simulink model "slide_mode_control"  (R2025b)
settings: Solver=ode23tb  StartTime=0.0  StopTime=t(end)  FixedStep=Ts  RelTol=1e-5
values from neighbouring files (symbols this model uses):
  alpha_0 = 0    [trajectory_smooth.m]
  beta_0 = 0    [trajectory_smooth.m]
  c = 40    [data.m]
  c1_inner = 15.0    (= 15)    [control_params.m]
  c1_outer = 5.0    (= 5)    [control_params.m]
  c1_swing = 8.5    [control_params.m]
  c2_inner = 4.5    [control_params.m]
  c2_outer = 7.5    [control_params.m]
  c2_swing = 5.5    [control_params.m]
  c_plant = c    (= 40)    [data.m]    (also in variation_params.m = scenarios(scen_idx, 2))
  cM = 1.779e-7    (= 1.779e-07)    [data.m]
  cT = 1.105e-5    (= 1.105e-05)    [data.m]
  d = 0.225    [data.m]
  d_alpha_0 = 0    [trajectory_smooth.m]
  d_beta_0 = 0    [trajectory_smooth.m]
  d_l_0 = 0    [trajectory_smooth.m]
  d_phi_0 = 0    [trajectory_smooth.m]
  d_psi_0 = dot_psi_d(1)    [trajectory_smooth.m]
  d_theta_0 = 0    [trajectory_smooth.m]
  d_x_0 = dot_csi_d(1, 1)    [trajectory_smooth.m]
  d_y_0 = dot_csi_d(2, 1)    [trajectory_smooth.m]
  d_z_0 = dot_csi_d(3, 1)    [trajectory_smooth.m]
  delta_val = 0.05    [control_params.m]
  epn_inner = 0.1    [control_params.m]
  epn_outer = 0.1    [control_params.m]
  epn_swing = 0.1    [control_params.m]
  Ixx = 0.0211    [data.m]
  Iyy = Ixx    (= 0.0211)    [data.m]
  Izz = 0.0366    [data.m]
  J_rp = 1.287e-4    (= 0.0001287)    [data.m]
  k = 1e5    (= 100000)    [data.m]
  k_inner = 15.0    (= 15)    [control_params.m]
  k_outer = 2.0    (= 2)    [control_params.m]
  k_plant = k    (= 100000)    [data.m]    (also in variation_params.m = scenarios(scen_idx, 1))
  k_swing = 10.0    (= 10)    [control_params.m]
  l_0 = L_rest + (m_plant*(g+ddot_csi_d(3,1)))/ k_plant    [trajectory_smooth.m]
  L_rest = 1    [data.m]
  M = 2    [data.m]
  m_plant = m    (= 0.5)    [data.m]    (also in variation_params.m = scenarios(scen_idx, 3))
  mu_1_inner = 5/3    (= 1.66666666667)    [control_params.m]
  mu_1_outer = 5/3    (= 1.66666666667)    [control_params.m]
  mu_1_swing = 5/3    (= 1.66666666667)    [control_params.m]
  mu_2_inner = 5/3    (= 1.66666666667)    [control_params.m]
  mu_2_outer = 5/3    (= 1.66666666667)    [control_params.m]
  mu_2_swing = 5/3    (= 1.66666666667)    [control_params.m]
  Omega_0 = w1_0 - w2_0 + w3_0 - w4_0    [trajectory_smooth.m]
  omega_n_1 = 20    [control_params.m]
  omega_n_2 = 20    [control_params.m]
  omega_square_0 = inv(A_alloc) * [u1_hover; u2_hover; u3_hover; u4_hover]    [trajectory_smooth.m]
  phi_0 = 0    [trajectory_smooth.m]
  psi_0 = psi_d(1)    [trajectory_smooth.m]
  theta_0 = 0    [trajectory_smooth.m]
  x_0 = csi_d(1, 1)    [trajectory_smooth.m]
  y_0 = csi_d(2, 1)    [trajectory_smooth.m]
  z_0 = csi_d(3, 1) + l_0    [trajectory_smooth.m]
  zeta_1 = 1    [control_params.m]
  zeta_2 = 1    [control_params.m]
settings Model: Creator=emanu  LastModifiedBy=emanu

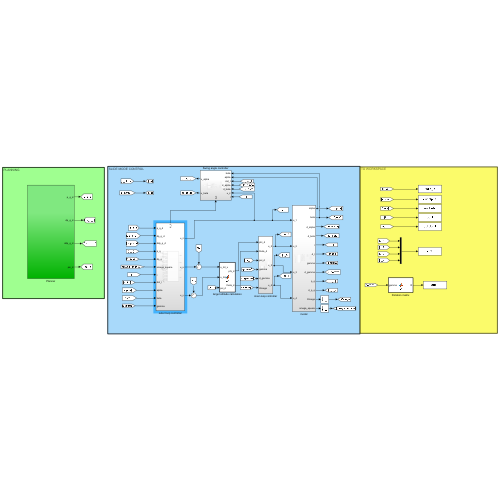
[thumbnail: Simulink's stored preview of the top-level diagram]
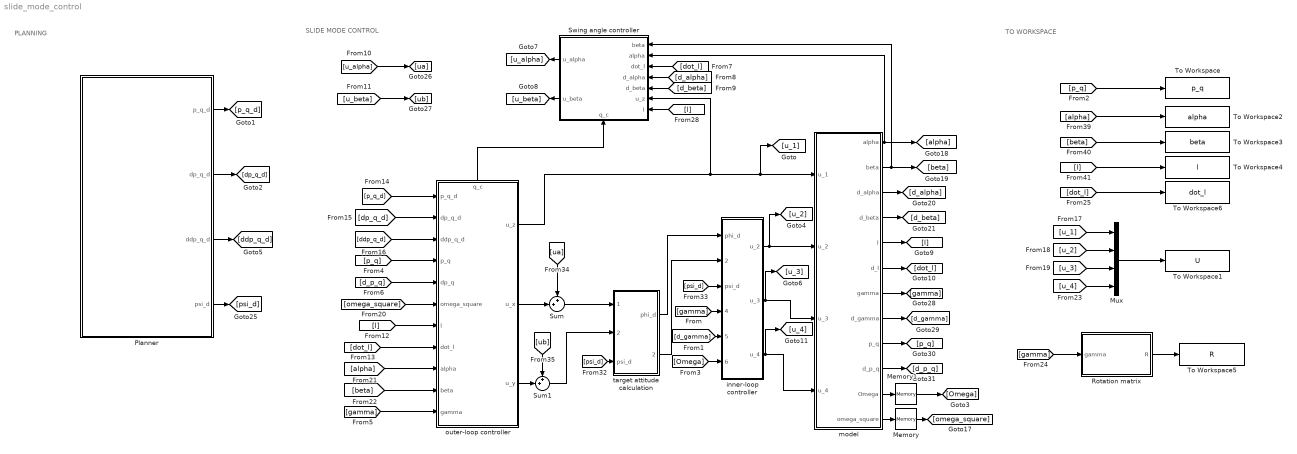
== system slide_mode_control ==
  note: PLANNING
  note: TO WORKSPACE
  note: SLIDE MODE CONTROL
  Memory : Memory  InitialCondition=omega_square_0
  Memory1 : Memory  InitialCondition=Omega_0
  Mux : Mux
  Planner : Subsystem
  Rotation matrix : MATLAB Function  TreatAsAtomicUnit=on
  Sum : Sum  Inputs=++|
  Sum1 : Sum  Inputs=++|
  Swing angle controller : Subsystem
      settings: PortSchema="{\"entries\":[{\"content\":{\"sides\":[{\"content\":{\"connectorIds\":[\"In1\",\"In2\",\"In3\",\"In4\",\"In5\",\"In6\",\"In7\"]},\"type\":\"ConnectorPlacement.EquallySpacedRectSide\",\"uuid\":\"107d9a79-5770-4fe1-afeb-f01ba17b8623\"},{\"content\":{\"connectorIds\":[\"Out1\",\"Out2\"],\"side\":\"RIGHT\"},\"type\":\"ConnectorPlacement.EquallySpacedRectSide\",\"uuid\":\"a16cfd03-53b4-494b-9a38-5d38c3257b94\"},{\"content\":{\"side\":\"TOP\"},\"type\":\"ConnectorPlacement.EquallySpacedRectSide\",\"uuid\":\"c63fb6e7-34b4-45e7-a650-d18239478a3a\"},{\"content\":{\"connectorIds\":[\"In8\"],\"side\":\"BOTTOM\"},\"type\":\"ConnectorPlacement.EquallySpacedRectSide\",\"uuid\":\"a663d818-4b24-4a2f-8491-f9b6658636ee\"}]},\"type\":\"ConnectorPlacement.EquallySpacedConnector\",\"uuid\":\"99174980-2348-474e-adfc-1c682a4a90eb\"}],\"packageUris\":[\"http://schema.mathworks.com/mf0/Connector/R2020b\"],\"version\":\"1.0\"}"
  To Workspace : ToWorkspace  VariableName=p_q  SaveFormat=Timeseries  SampleTime=-1
  To Workspace1 : ToWorkspace  VariableName=U  SaveFormat=Timeseries  SampleTime=-1
  To Workspace2 : ToWorkspace  VariableName=alpha  SaveFormat=Timeseries  SampleTime=-1
  To Workspace3 : ToWorkspace  VariableName=beta  SaveFormat=Timeseries  SampleTime=-1
  To Workspace4 : ToWorkspace  VariableName=l  SaveFormat=Timeseries  SampleTime=-1
  To Workspace5 : ToWorkspace  VariableName=R  SaveFormat=Timeseries  SampleTime=-1
  To Workspace6 : ToWorkspace  VariableName=dot_l  SaveFormat=Timeseries  SampleTime=-1
  inner-loop controller : Subsystem
  model : Subsystem
  outer-loop controller : Subsystem
      settings: PortSchema="{\"entries\":[{\"content\":{\"sides\":[{\"content\":{\"connectorIds\":[\"In1\",\"In2\",\"In3\",\"In4\",\"In5\",\"In6\",\"In7\",\"In8\",\"In9\",\"In10\",\"In11\"]},\"type\":\"ConnectorPlacement.EquallySpacedRectSide\",\"uuid\":\"df6fcbf3-dc8d-434b-9cb1-436330819ec6\"},{\"content\":{\"connectorIds\":[\"Out1\",\"Out2\",\"Out3\"],\"side\":\"RIGHT\"},\"type\":\"ConnectorPlacement.EquallySpacedRectSide\",\"uuid\":\"251502b7-b7f3-4a5f-b6bf-a36f68ad90ea\"},{\"content\":{\"connectorIds\":[\"Out4\"],\"side\":\"TOP\"},\"type\":\"ConnectorPlacement.EquallySpacedRectSide\",\"uuid\":\"43b3d9fa-4196-44c6-9465-37a7290486e2\"}]},\"type\":\"ConnectorPlacement.EquallySpacedConnector\",\"uuid\":\"0c84f21f-ead6-4ba1-8038-c5609232fb5a\"}],\"packageUris\":[\"http://schema.mathworks.com/mf0/Connector/R2020b\"],\"version\":\"1.0\"}"
  target attitude calculation : MATLAB Function  TreatAsAtomicUnit=on
  wires:
  [Omega] -> inner-loop controller/6(Omega)
  outer-loop controller/2(u_x) -> Sum/2
  outer-loop controller/3(u_y) -> Sum1/2
  Swing angle controller/1(u_alpha) -> [u_alpha]
  Swing angle controller/2(u_beta) -> [u_beta]
  Sum1/1 -> target attitude calculation/2(u_tot_y)
  Sum/1 -> target attitude calculation/1(u_tot_x)
  target attitude calculation/2(theta_d) -> inner-loop controller/2(theta_d)
  target attitude calculation/1(phi_d) -> inner-loop controller/1(phi_d)
  inner-loop controller/1(u_2) -> [u_2], model/2(u_2)
  inner-loop controller/2(u_3) -> model/3(u_3), [u_3]
  inner-loop controller/3(u_4) -> model/4(u_4), [u_4]
  outer-loop controller/1(u_z) -> Swing angle controller/6(u_z), [u_1], model/1(u_1)
  Memory/1 -> [omega_square]
  Memory1/1 -> [Omega]
  [dot_l] -> Swing angle controller/3(dot_l)
  [d_alpha] -> Swing angle controller/4(d_alpha)
  [d_beta] -> Swing angle controller/5(d_beta)
  [l] -> Swing angle controller/7(l)
  Planner/4(psi_d) -> [psi_d]
  [psi_d] -> target attitude calculation/3(psi_d)
  [u_beta] -> [ub]
  [u_alpha] -> [ua]
  [ua] -> Sum/1
  [ub] -> Sum1/1
  [beta] -> To Workspace3/1
  [alpha] -> To Workspace2/1
  [l] -> To Workspace4/1
  model/1(alpha) -> Swing angle controller/2(alpha), [alpha]
  model/2(beta) -> Swing angle controller/1(beta), [beta]
  model/3(d_alpha) -> [d_alpha]
  model/4(d_beta) -> [d_beta]
  model/6(d_l) -> [dot_l]
  model/5(l) -> [l]
  model/11(Omega) -> Memory1/1
  model/12(omega_square) -> Memory/1
  model/7(gamma) -> [gamma]
  model/9(p_q) -> [p_q]
  model/10(d_p_q) -> [d_p_q]
  model/8(d_gamma) -> [d_gamma]
  [psi_d] -> inner-loop controller/3(psi_d)
  [gamma] -> inner-loop controller/4(gamma)
  [d_gamma] -> inner-loop controller/5(d_gamma)
  [p_q] -> To Workspace/1
  [omega_square] -> outer-loop controller/6(omega_square)
  [l] -> outer-loop controller/7(l)
  [dot_l] -> outer-loop controller/8(dot_l)
  [alpha] -> outer-loop controller/9(alpha)
  [beta] -> outer-loop controller/10(beta)
  [gamma] -> outer-loop controller/11(gamma)
  [p_q] -> outer-loop controller/4(p_q)
  [d_p_q] -> outer-loop controller/5(dp_q)
  Planner/1(p_q_d) -> [p_q_d]
  [p_q_d] -> outer-loop controller/1(p_q_d)
  Planner/2(dp_q_d) -> [dp_q_d]
  [dp_q_d] -> outer-loop controller/2(dp_q_d)
  Planner/3(ddp_q_d) -> [ddp_q_d]
  [ddp_q_d] -> outer-loop controller/3(ddp_q_d)
  [u_1] -> Mux/1
  [u_2] -> Mux/2
  [u_3] -> Mux/3
  [u_4] -> Mux/4
  Mux/1 -> To Workspace1/1
  [gamma] -> Rotation matrix/1(gamma)
  Rotation matrix/1(R) -> To Workspace5/1
  [dot_l] -> To Workspace6/1
  outer-loop controller/4(q_c) -> Swing angle controller/8(q_c)

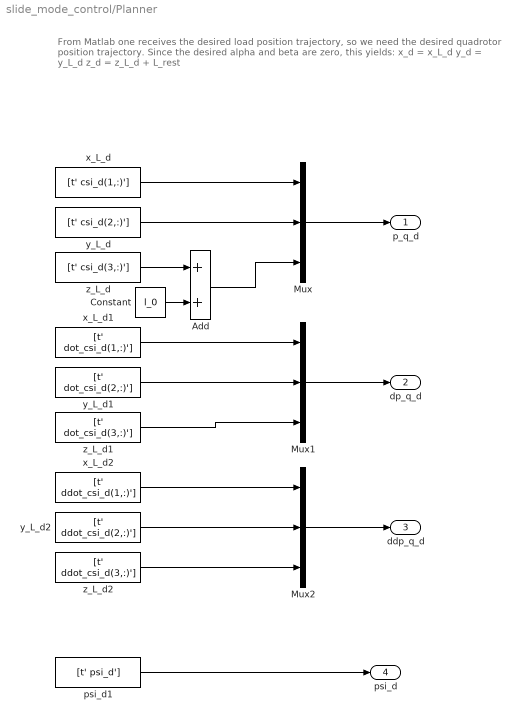
== system slide_mode_control/Planner ==
  note: From Matlab one receives the desired load position trajectory, so we need the desired quadrotor position trajectory. Since the desired alpha and beta are zero, this yields:
      | x_d = x_L_d
      | y_d = y_L_d
      | z_d = z_L_d + L_rest
  Add : Sum
  Constant : Constant  Value=l_0
  Mux : Mux  Inputs=3
  Mux1 : Mux  Inputs=3
  Mux2 : Mux  Inputs=3
  psi_d1 : FromWorkspace  VariableName=[t' psi_d']  OutputAfterFinalValue=Holding final value
  x_L_d : FromWorkspace  VariableName=[t' csi_d(1,:)']  OutputAfterFinalValue=Holding final value
  x_L_d1 : FromWorkspace  VariableName=[t' dot_csi_d(1,:)']  OutputAfterFinalValue=Setting to zero
  x_L_d2 : FromWorkspace  VariableName=[t' ddot_csi_d(1,:)']  OutputAfterFinalValue=Setting to zero
  y_L_d : FromWorkspace  VariableName=[t' csi_d(2,:)']  OutputAfterFinalValue=Holding final value
  y_L_d1 : FromWorkspace  VariableName=[t' dot_csi_d(2,:)']  OutputAfterFinalValue=Setting to zero
  y_L_d2 : FromWorkspace  VariableName=[t' ddot_csi_d(2,:)']  OutputAfterFinalValue=Setting to zero
  z_L_d : FromWorkspace  VariableName=[t' csi_d(3,:)']  OutputAfterFinalValue=Holding final value
  z_L_d1 : FromWorkspace  VariableName=[t' dot_csi_d(3,:)']  OutputAfterFinalValue=Setting to zero
  z_L_d2 : FromWorkspace  VariableName=[t' ddot_csi_d(3,:)']  OutputAfterFinalValue=Holding final value
  p_q_d : Outport
  dp_q_d : Outport  Port=2
  ddp_q_d : Outport  Port=3
  psi_d : Outport  Port=4
  wires:
  z_L_d/1 -> Add/1
  psi_d1/1 -> psi_d/1
  Constant/1 -> Add/2
  Add/1 -> Mux/3
  y_L_d/1 -> Mux/2
  x_L_d/1 -> Mux/1
  Mux/1 -> p_q_d/1
  x_L_d1/1 -> Mux1/1
  y_L_d1/1 -> Mux1/2
  z_L_d2/1 -> Mux2/3
  y_L_d2/1 -> Mux2/2
  x_L_d2/1 -> Mux2/1
  z_L_d1/1 -> Mux1/3
  Mux2/1 -> ddp_q_d/1
  Mux1/1 -> dp_q_d/1

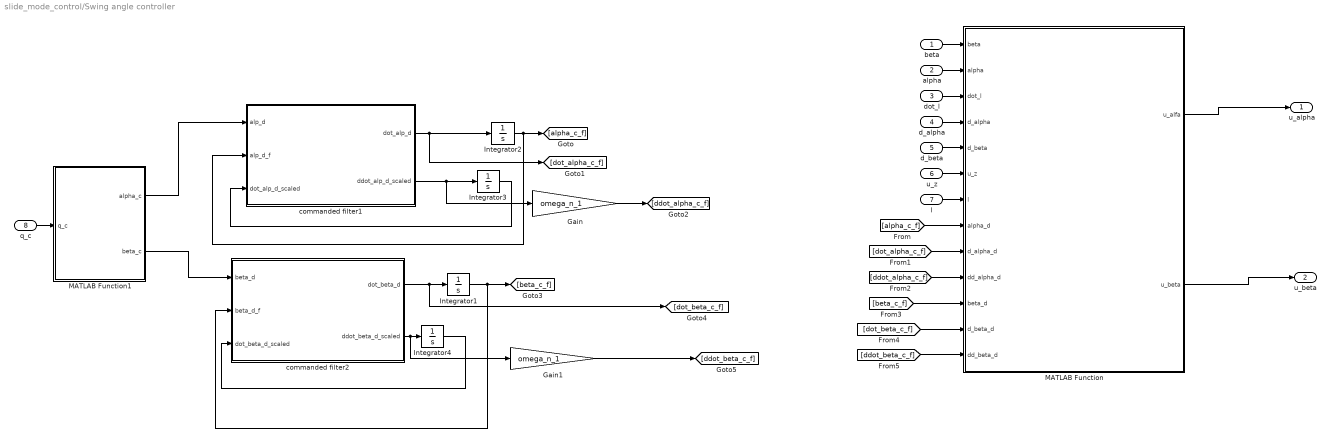
== system slide_mode_control/Swing angle controller ==
  beta : Inport
  alpha : Inport  Port=2
  dot_l : Inport  Port=3
  d_alpha : Inport  Port=4
  d_beta : Inport  Port=5
  u_z : Inport  Port=6
  l : Inport  Port=7
  q_c : Inport  Port=8
  Gain : Gain  Gain=omega_n_1
  Gain1 : Gain  Gain=omega_n_1
  Integrator1 : Integrator  InitialCondition=beta_0
  Integrator2 : Integrator  InitialCondition=alpha_0
  Integrator3 : Integrator  InitialCondition=d_alpha_0
  Integrator4 : Integrator  InitialCondition=d_beta_0
  MATLAB Function : MATLAB Function  TreatAsAtomicUnit=on
  MATLAB Function1 : MATLAB Function  TreatAsAtomicUnit=on
  commanded filter1 : MATLAB Function  TreatAsAtomicUnit=on
  commanded filter2 : MATLAB Function  TreatAsAtomicUnit=on
  u_alpha : Outport
  u_beta : Outport  Port=2
  wires:
  MATLAB Function/1(u_alfa) -> u_alpha/1
  MATLAB Function/2(u_beta) -> u_beta/1
  beta/1 -> MATLAB Function/1(beta)
  alpha/1 -> MATLAB Function/2(alpha)
  dot_l/1 -> MATLAB Function/3(dot_l)
  d_alpha/1 -> MATLAB Function/4(d_alpha)
  d_beta/1 -> MATLAB Function/5(d_beta)
  u_z/1 -> MATLAB Function/6(u_z)
  l/1 -> MATLAB Function/7(l)
  q_c/1 -> MATLAB Function1/1(q_c)
  commanded filter2/1(dot_beta_d) -> [dot_beta_c_f], Integrator1/1
  commanded filter1/1(dot_alp_d) -> [dot_alpha_c_f], Integrator2/1
  commanded filter1/2(ddot_alp_d_scaled) -> Gain/1, Integrator3/1
  Integrator2/1 -> [alpha_c_f], commanded filter1/2(alp_d_f)
  Gain1/1 -> [ddot_beta_c_f]
  Integrator4/1 -> commanded filter2/3(dot_beta_d_scaled)
  commanded filter2/2(ddot_beta_d_scaled) -> Integrator4/1, Gain1/1
  Integrator3/1 -> commanded filter1/3(dot_alp_d_scaled)
  Gain/1 -> [ddot_alpha_c_f]
  MATLAB Function1/1(alpha_c) -> commanded filter1/1(alp_d)
  Integrator1/1 -> [beta_c_f], commanded filter2/2(beta_d_f)
  MATLAB Function1/2(beta_c) -> commanded filter2/1(beta_d)
  [alpha_c_f] -> MATLAB Function/8(alpha_d)
  [dot_alpha_c_f] -> MATLAB Function/9(d_alpha_d)
  [ddot_alpha_c_f] -> MATLAB Function/10(dd_alpha_d)
  [beta_c_f] -> MATLAB Function/11(beta_d)
  [dot_beta_c_f] -> MATLAB Function/12(d_beta_d)
  [ddot_beta_c_f] -> MATLAB Function/13(dd_beta_d)

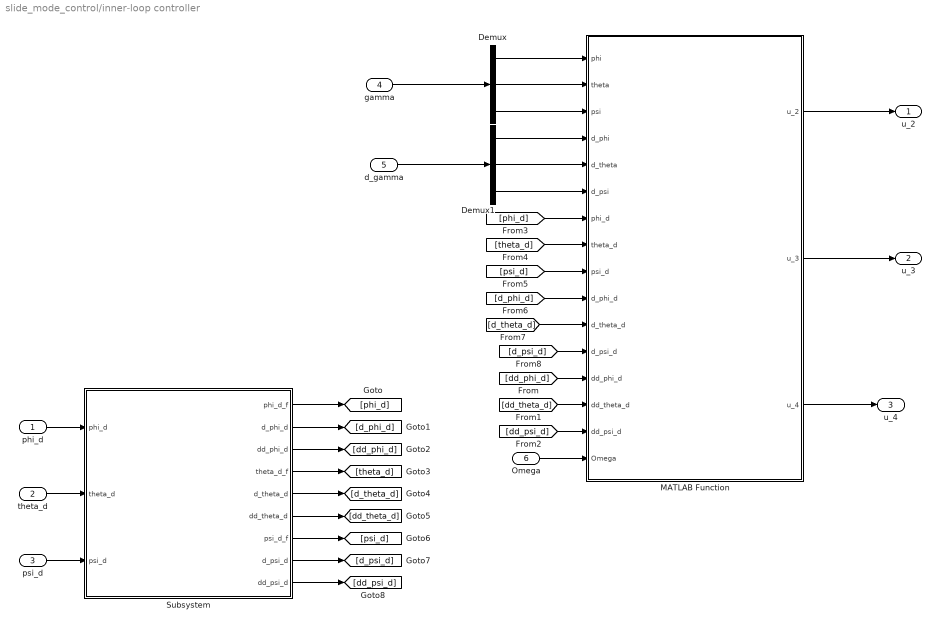
== system slide_mode_control/inner-loop controller ==
  phi_d : Inport
  theta_d : Inport  Port=2
  psi_d : Inport  Port=3
  gamma : Inport  Port=4
  d_gamma : Inport  Port=5
  Omega : Inport  Port=6
  Demux : Demux  Outputs=3
  Demux1 : Demux  Outputs=3
  MATLAB Function : MATLAB Function  TreatAsAtomicUnit=on
  Subsystem : Subsystem
  u_2 : Outport
  u_3 : Outport  Port=2
  u_4 : Outport  Port=3
  wires:
  phi_d/1 -> Subsystem/1(phi_d)
  theta_d/1 -> Subsystem/2(theta_d)
  psi_d/1 -> Subsystem/3(psi_d)
  Subsystem/1(phi_d_f) -> [phi_d]
  Subsystem/2(d_phi_d) -> [d_phi_d]
  Subsystem/3(dd_phi_d) -> [dd_phi_d]
  Subsystem/4(theta_d_f) -> [theta_d]
  Subsystem/5(d_theta_d) -> [d_theta_d]
  Subsystem/6(dd_theta_d) -> [dd_theta_d]
  Subsystem/7(psi_d_f) -> [psi_d]
  Subsystem/8(d_psi_d) -> [d_psi_d]
  Subsystem/9(dd_psi_d) -> [dd_psi_d]
  Omega/1 -> MATLAB Function/16(Omega)
  MATLAB Function/1(u_2) -> u_2/1
  MATLAB Function/2(u_3) -> u_3/1
  MATLAB Function/3(u_4) -> u_4/1
  [dd_phi_d] -> MATLAB Function/13(dd_phi_d)
  [dd_theta_d] -> MATLAB Function/14(dd_theta_d)
  [dd_psi_d] -> MATLAB Function/15(dd_psi_d)
  [d_phi_d] -> MATLAB Function/10(d_phi_d)
  [d_theta_d] -> MATLAB Function/11(d_theta_d)
  [d_psi_d] -> MATLAB Function/12(d_psi_d)
  [phi_d] -> MATLAB Function/7(phi_d)
  [theta_d] -> MATLAB Function/8(theta_d)
  [psi_d] -> MATLAB Function/9(psi_d)
  gamma/1 -> Demux/1
  Demux/1 -> MATLAB Function/1(phi)
  Demux/2 -> MATLAB Function/2(theta)
  Demux/3 -> MATLAB Function/3(psi)
  Demux1/1 -> MATLAB Function/4(d_phi)
  Demux1/2 -> MATLAB Function/5(d_theta)
  Demux1/3 -> MATLAB Function/6(d_psi)
  d_gamma/1 -> Demux1/1

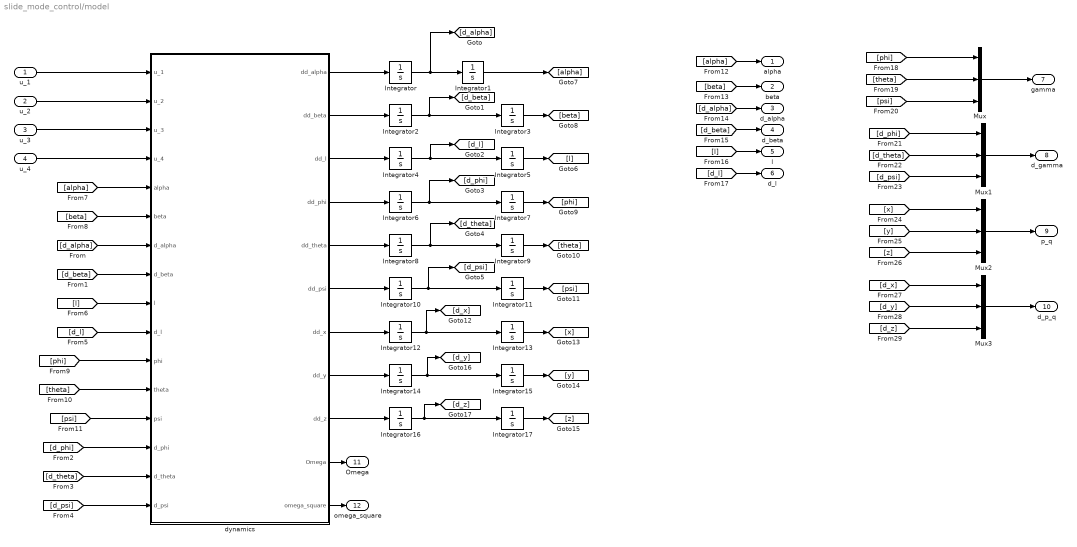
== system slide_mode_control/model ==
  u_1 : Inport
  u_2 : Inport  Port=2
  u_3 : Inport  Port=3
  u_4 : Inport  Port=4
  Integrator : Integrator  InitialCondition=d_alpha_0
  Integrator1 : Integrator  InitialCondition=alpha_0
  Integrator10 : Integrator  InitialCondition=d_psi_0
  Integrator11 : Integrator  InitialCondition=psi_0
  Integrator12 : Integrator  InitialCondition=d_x_0
  Integrator13 : Integrator  InitialCondition=x_0
  Integrator14 : Integrator  InitialCondition=d_y_0
  Integrator15 : Integrator  InitialCondition=y_0
  Integrator16 : Integrator  InitialCondition=d_z_0
  Integrator17 : Integrator  InitialCondition=z_0
  Integrator2 : Integrator  InitialCondition=d_beta_0
  Integrator3 : Integrator  InitialCondition=beta_0
  Integrator4 : Integrator  InitialCondition=d_l_0
  Integrator5 : Integrator  InitialCondition=l_0
  Integrator6 : Integrator  InitialCondition=d_phi_0
  Integrator7 : Integrator  InitialCondition=phi_0
  Integrator8 : Integrator  InitialCondition=d_theta_0
  Integrator9 : Integrator  InitialCondition=theta_0
  Mux{,1..3} (4 alike) : Mux  Inputs=3
  dynamics : MATLAB Function  TreatAsAtomicUnit=on
  alpha : Outport
  beta : Outport  Port=2
  d_alpha : Outport  Port=3
  d_beta : Outport  Port=4
  l : Outport  Port=5
  d_l : Outport  Port=6
  gamma : Outport  Port=7
  d_gamma : Outport  Port=8
  p_q : Outport  Port=9
  d_p_q : Outport  Port=10
  Omega : Outport  Port=11
  omega_square : Outport  Port=12
  wires:
  dynamics/1(dd_alpha) -> Integrator/1
  Integrator/1 -> [d_alpha], Integrator1/1
  dynamics/2(dd_beta) -> Integrator2/1
  Integrator2/1 -> [d_beta], Integrator3/1
  dynamics/3(dd_l) -> Integrator4/1
  dynamics/4(dd_phi) -> Integrator6/1
  dynamics/5(dd_theta) -> Integrator8/1
  Integrator4/1 -> [d_l], Integrator5/1
  Integrator6/1 -> [d_phi], Integrator7/1
  Integrator8/1 -> [d_theta], Integrator9/1
  dynamics/6(dd_psi) -> Integrator10/1
  Integrator10/1 -> [d_psi], Integrator11/1
  dynamics/7(dd_x) -> Integrator12/1
  Integrator12/1 -> [d_x], Integrator13/1
  dynamics/8(dd_y) -> Integrator14/1
  dynamics/9(dd_z) -> Integrator16/1
  Integrator14/1 -> [d_y], Integrator15/1
  Integrator16/1 -> [d_z], Integrator17/1
  [d_alpha] -> dynamics/7(d_alpha)
  [d_beta] -> dynamics/8(d_beta)
  [d_phi] -> dynamics/14(d_phi)
  [d_theta] -> dynamics/15(d_theta)
  [d_psi] -> dynamics/16(d_psi)
  [d_l] -> dynamics/10(d_l)
  Integrator5/1 -> [l]
  [l] -> dynamics/9(l)
  Integrator1/1 -> [alpha]
  Integrator3/1 -> [beta]
  [alpha] -> dynamics/5(alpha)
  [beta] -> dynamics/6(beta)
  u_1/1 -> dynamics/1(u_1)
  u_2/1 -> dynamics/2(u_2)
  u_3/1 -> dynamics/3(u_3)
  u_4/1 -> dynamics/4(u_4)
  Integrator11/1 -> [psi]
  Integrator13/1 -> [x]
  Integrator17/1 -> [z]
  dynamics/10(Omega) -> Omega/1
  dynamics/11(omega_square) -> omega_square/1
  [theta] -> dynamics/12(theta)
  [psi] -> dynamics/13(psi)
  [phi] -> dynamics/11(phi)
  Integrator7/1 -> [phi]
  Integrator9/1 -> [theta]
  Integrator15/1 -> [y]
  [alpha] -> alpha/1
  [beta] -> beta/1
  [d_alpha] -> d_alpha/1
  [d_beta] -> d_beta/1
  [l] -> l/1
  [d_l] -> d_l/1
  [phi] -> Mux/1
  [theta] -> Mux/2
  [psi] -> Mux/3
  Mux/1 -> gamma/1
  Mux1/1 -> d_gamma/1
  [d_psi] -> Mux1/3
  [d_theta] -> Mux1/2
  [d_phi] -> Mux1/1
  [x] -> Mux2/1
  [y] -> Mux2/2
  [z] -> Mux2/3
  Mux2/1 -> p_q/1
  Mux3/1 -> d_p_q/1
  [d_z] -> Mux3/3
  [d_y] -> Mux3/2
  [d_x] -> Mux3/1

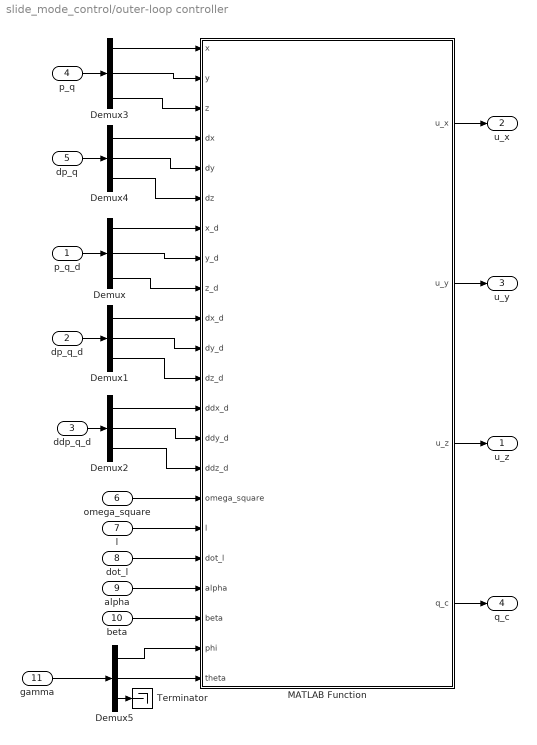
== system slide_mode_control/outer-loop controller ==
  p_q_d : Inport
  dp_q_d : Inport  Port=2
  ddp_q_d : Inport  Port=3
  p_q : Inport  Port=4
  dp_q : Inport  Port=5
  omega_square : Inport  Port=6
  l : Inport  Port=7
  dot_l : Inport  Port=8
  alpha : Inport  Port=9
  beta : Inport  Port=10
  gamma : Inport  Port=11
  Demux{,1..5} (6 alike) : Demux  Outputs=3
  MATLAB Function : MATLAB Function  TreatAsAtomicUnit=on
  Terminator : Terminator
  u_z : Outport
  u_x : Outport  Port=2
  u_y : Outport  Port=3
  q_c : Outport  Port=4
  wires:
  MATLAB Function/1(u_x) -> u_x/1
  MATLAB Function/2(u_y) -> u_y/1
  MATLAB Function/3(u_z) -> u_z/1
  omega_square/1 -> MATLAB Function/16(omega_square)
  l/1 -> MATLAB Function/17(l)
  dot_l/1 -> MATLAB Function/18(dot_l)
  alpha/1 -> MATLAB Function/19(alpha)
  beta/1 -> MATLAB Function/20(beta)
  p_q_d/1 -> Demux/1
  Demux/1 -> MATLAB Function/7(x_d)
  Demux/2 -> MATLAB Function/8(y_d)
  Demux/3 -> MATLAB Function/9(z_d)
  dp_q_d/1 -> Demux1/1
  Demux1/1 -> MATLAB Function/10(dx_d)
  Demux1/2 -> MATLAB Function/11(dy_d)
  Demux1/3 -> MATLAB Function/12(dz_d)
  ddp_q_d/1 -> Demux2/1
  Demux2/1 -> MATLAB Function/13(ddx_d)
  Demux2/2 -> MATLAB Function/14(ddy_d)
  Demux2/3 -> MATLAB Function/15(ddz_d)
  p_q/1 -> Demux3/1
  Demux3/1 -> MATLAB Function/1(x)
  Demux3/2 -> MATLAB Function/2(y)
  Demux3/3 -> MATLAB Function/3(z)
  dp_q/1 -> Demux4/1
  Demux4/1 -> MATLAB Function/4(dx)
  Demux4/2 -> MATLAB Function/5(dy)
  Demux4/3 -> MATLAB Function/6(dz)
  Demux5/3 -> Terminator/1
  gamma/1 -> Demux5/1
  Demux5/1 -> MATLAB Function/21(phi)
  Demux5/2 -> MATLAB Function/22(theta)
  MATLAB Function/4(q_c) -> q_c/1

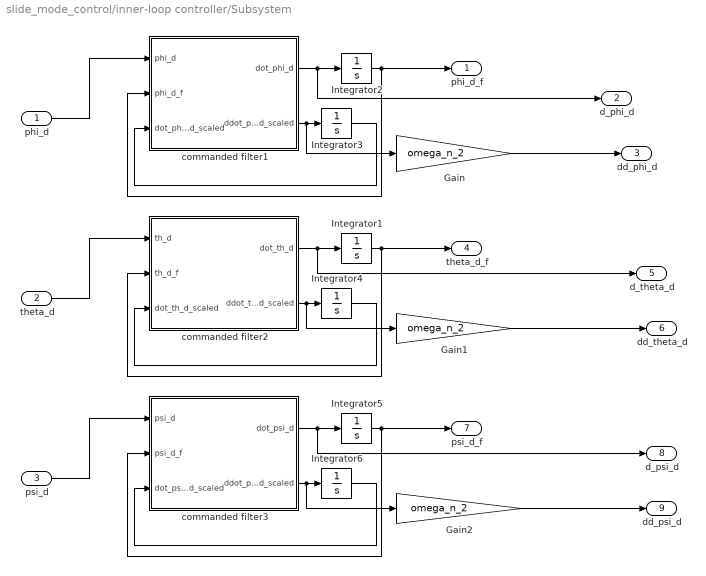
== system slide_mode_control/inner-loop controller/Subsystem ==
  phi_d : Inport
  theta_d : Inport  Port=2
  psi_d : Inport  Port=3
  Gain : Gain  Gain=omega_n_2
  Gain1 : Gain  Gain=omega_n_2
  Gain2 : Gain  Gain=omega_n_2
  Integrator1 : Integrator  InitialCondition=theta_0
  Integrator2 : Integrator  InitialCondition=phi_0
  Integrator3 : Integrator  InitialCondition=d_phi_0
  Integrator4 : Integrator  InitialCondition=d_theta_0
  Integrator5 : Integrator  InitialCondition=psi_0
  Integrator6 : Integrator  InitialCondition=d_psi_0
  commanded filter1 : MATLAB Function  TreatAsAtomicUnit=on
  commanded filter2 : MATLAB Function  TreatAsAtomicUnit=on
  commanded filter3 : MATLAB Function  TreatAsAtomicUnit=on
  phi_d_f : Outport
  d_phi_d : Outport  Port=2
  dd_phi_d : Outport  Port=3
  theta_d_f : Outport  Port=4
  d_theta_d : Outport  Port=5
  dd_theta_d : Outport  Port=6
  psi_d_f : Outport  Port=7
  d_psi_d : Outport  Port=8
  dd_psi_d : Outport  Port=9
  wires:
  phi_d/1 -> commanded filter1/1(phi_d)
  commanded filter1/1(dot_phi_d) -> d_phi_d/1, Integrator2/1
  Integrator2/1 -> phi_d_f/1, commanded filter1/2(phi_d_f)
  Integrator3/1 -> commanded filter1/3(dot_phi_d_scaled)
  commanded filter1/2(ddot_phi_d_scaled) -> Gain/1, Integrator3/1
  Gain/1 -> dd_phi_d/1
  Gain1/1 -> dd_theta_d/1
  commanded filter2/2(ddot_th_d_scaled) -> Gain1/1, Integrator4/1
  Integrator1/1 -> theta_d_f/1, commanded filter2/2(th_d_f)
  Integrator4/1 -> commanded filter2/3(dot_th_d_scaled)
  theta_d/1 -> commanded filter2/1(th_d)
  commanded filter2/1(dot_th_d) -> d_theta_d/1, Integrator1/1
  Gain2/1 -> dd_psi_d/1
  commanded filter3/2(ddot_psi_d_scaled) -> Gain2/1, Integrator6/1
  Integrator5/1 -> psi_d_f/1, commanded filter3/2(psi_d_f)
  Integrator6/1 -> commanded filter3/3(dot_psi_d_scaled)
  psi_d/1 -> commanded filter3/1(psi_d)
  commanded filter3/1(dot_psi_d) -> d_psi_d/1, Integrator5/1

== matlab function slide_mode_control/inner-loop controller/Subsystem/commanded filter2 ==
  data: th_d input; dot_th_d output; th_d_f input; dot_th_d_scaled input; zeta_2 parameter; ddot_th_d_scaled output; omega_n_2 parameter
function [dot_th_d, ddot_th_d_scaled] = fcn(th_d, th_d_f, dot_th_d_scaled, zeta_2, omega_n_2)
    dot_th_d = omega_n_2 * dot_th_d_scaled;
    ddot_th_d_scaled = -2 * zeta_2 * omega_n_2 * dot_th_d_scaled - omega_n_2 * (th_d_f - th_d);
end

== matlab function slide_mode_control/inner-loop controller/Subsystem/commanded filter3 ==
  data: psi_d input; dot_psi_d output; psi_d_f input; dot_psi_d_scaled input; zeta_2 parameter; ddot_psi_d_scaled output; omega_n_2 parameter
function [dot_psi_d, ddot_psi_d_scaled] = fcn(psi_d, psi_d_f, dot_psi_d_scaled, zeta_2, omega_n_2)
    dot_psi_d = omega_n_2 * dot_psi_d_scaled;
    ddot_psi_d_scaled = -2 * zeta_2 * omega_n_2 * dot_psi_d_scaled - omega_n_2 * (psi_d_f - psi_d);
end

== matlab function slide_mode_control/Swing angle controller/MATLAB Function ==
  data: beta input; u_alfa output; u_beta output; alpha input; dot_l input; d_alpha input; d_beta input; u_z input; l input; alpha_d input; d_alpha_d input; dd_alpha_d input; beta_d input; d_beta_d input; dd_beta_d input; M parameter; c1_swing parameter; c2_swing parameter; k_swing parameter; mu_1_swing parameter; mu_2_swing parameter; epn_swing parameter; delta_val parameter
function [u_alfa, u_beta] = fcn(beta, alpha, dot_l, d_alpha, d_beta, u_z, l,alpha_d,d_alpha_d,dd_alpha_d, ...
    beta_d,d_beta_d,dd_beta_d, M,c1_swing, c2_swing,k_swing,mu_1_swing, mu_2_swing, epn_swing, delta_val)
    L = max(l, 1e-3);
    cos_beta = max(cos(beta), 1e-3);
    eps_g = 1e-4;

    g_alfa = -u_z / (M * L * cos_beta);
    g_beta =  -u_z / (M * L);

    f_alfa = -2 * (dot_l * d_alpha / L) + 2 * d_alpha * d_beta * (sin(beta) / cos_beta);
    f_beta = -2 * (dot_l * d_beta / L) - d_alpha^2 * sin(beta) * cos_beta;

    % surface parameters
    c1 = c1_swing; 
    c2 =c2_swing; 
    mu_1 = mu_1_swing; 
    mu_2 = mu_2_swing; 
    epn = epn_swing;

    % Errors
    e_alfa = alpha_d-alpha;
    dot_e_alfa = d_alpha_d-d_alpha;
    e_beta = beta_d-beta;
    dot_e_beta = d_beta_d-d_beta;

  
    s_alfa = e_alfa + c1 * sign(e_alfa) * abs(e_alfa)^mu_1 + c2 * sign(dot_e_alfa) * abs(dot_e_alfa)^mu_2;
    s_beta = e_beta + c1 * sign(e_beta) * abs(e_beta)^mu_1 + c2 * sign(dot_e_beta) * abs(dot_e_beta)^mu_2;

    delta=delta_val;

    num_a = (sign(dot_e_alfa) * abs(dot_e_alfa)^(2-mu_2) / (c2 * mu_2)) * (1 + c1 * mu_1 * abs(e_alfa)^(mu_1-1))+dd_alpha_d- f_alfa + k_swing * s_alfa + epn * sat(s_alfa, delta);
    num_b = (sign(dot_e_beta) * abs(dot_e_beta)^(2-mu_2) / (c2 * mu_2)) * (1 + c1 * mu_1 * abs(e_beta)^(mu_1-1))+dd_beta_d- f_beta + k_swing * s_beta + epn * sat(s_beta, delta);


    if abs(g_alfa) < eps_g
        u_alfa = num_a / (sign(g_alfa + eps) * eps_g);
    else
        u_alfa = num_a / g_alfa;
    end

    if abs(g_beta) < eps_g
        u_beta = num_b / (sign(g_beta + eps) * eps_g);
    else
        u_beta = num_b / g_beta;
    end
end

== matlab function slide_mode_control/outer-loop controller/MATLAB Function ==
  data: u_x output; u_y output; u_z output; x input; y input; z input; dx input; dy input; dz input; x_d input; y_d input; z_d input; dx_d input; dy_d input; dz_d input; ddx_d input; ddy_d input; ddz_d input; omega_square input; k parameter; L_rest parameter; c parameter; l input; dot_l input; alpha input; beta input; M parameter; phi input; theta input; cT parameter; c1_outer parameter; c2_outer parameter; k_outer parameter; mu_1_outer parameter; mu_2_outer parameter; epn_outer parameter; delta_val parameter; q_c output size=3
function [u_x, u_y, u_z,q_c] = fcn(x, y, z, dx, dy, dz,x_d,y_d,z_d,dx_d,dy_d,dz_d, ddx_d, ddy_d, ddz_d, ...
    omega_square, k, L_rest, c, l, dot_l, alpha, beta, M, phi, theta, cT,c1_outer, c2_outer,k_outer, ...
    mu_1_outer, mu_2_outer, epn_outer, delta_val)

T=k*(l-L_rest)+c*dot_l;
Tx=T*sin(alpha)*cos(beta);
Ty=T*sin(beta);
Tz=T*cos(alpha)*cos(beta);
g=9.81;

F=max((cT*sum(omega_square)),1e-3);
cos_phi_theta=max((cos(phi)*cos(theta)), 1e-3);


g_x=F/M;
g_y=g_x;
g_z=cos_phi_theta/M;

f_x=-Tx/M;
f_y=-Ty/M;
f_z=-(Tz/M)-g;

%parameter surface
c1 = c1_outer;
c2 = c2_outer;
mu_1 = mu_1_outer;
mu_2 = mu_2_outer;
epn=epn_outer;

%error
ex=x_d-x;
ey=y_d-y;
ez=z_d-z;
dex=dx_d-dx;
dey=dy_d-dy;
dez=dz_d-dz;

%surface
s_x = ex + c1 * sign(ex) * abs(ex)^mu_1 + c2 * sign(dex) * abs(dex)^mu_2;
s_y = ey + c1 * sign(ey) * abs(ey)^mu_1 + c2 * sign(dey) * abs(dey)^mu_2;
s_z = ez + c1 * sign(ez) * abs(ez)^mu_1 + c2 * sign(dez) * abs(dez)^mu_2;

delta=delta_val;

num_x = (sign(dex) * abs(dex)^(2 - mu_2) / (c2 * mu_2)) * (1 + c1 * mu_1 * abs(ex)^(mu_1 - 1)) + ddx_d - f_x + k_outer * s_x + epn * sat(s_x, delta); 
num_y = (sign(dey) * abs(dey)^(2 - mu_2) / (c2 * mu_2)) * (1 + c1 * mu_1 * abs(ey)^(mu_1 - 1)) + ddy_d - f_y + k_outer * s_y + epn * sat(s_y, delta); 
num_z = (sign(dez) * abs(dez)^(2 - mu_2) / (c2 * mu_2)) * (1 + c1 * mu_1 * abs(ez)^(mu_1 - 1)) + ddz_d - f_z + k_outer * s_z + epn * sat(s_z, delta); 

u_x=num_x/g_x;
u_y=num_y/g_y;
u_z=num_z/g_z;

u_des=[num_x;num_y;num_z];

if norm(u_des)<1e-5
    q_c=[0;0;-1];
else
    q_c=-u_des/norm(u_des);
end

end

== matlab function slide_mode_control/Rotation matrix ==
  data: gamma input; R output
function R = fcn(gamma)

phi=gamma(1);
theta=gamma(2);
psi=gamma(3);

c_phi = cos(phi);   s_phi = sin(phi);
c_the = cos(theta); s_the = sin(theta);
c_psi = cos(psi);   s_psi = sin(psi);

% R_B^E (Z-Y-X Euler angles)
R = [ c_the*c_psi,  s_phi*s_the*c_psi - c_phi*s_psi,  c_phi*s_the*c_psi + s_phi*s_psi;
      c_the*s_psi,  s_phi*s_the*s_psi + c_phi*c_psi,  c_phi*s_the*s_psi - s_phi*c_psi;
     -s_the,        s_phi*c_the,                      c_phi*c_the ];
end

== matlab function slide_mode_control/Swing angle controller/MATLAB Function1 ==
  data: q_c input size=3; alpha_c output; beta_c output
function [alpha_c, beta_c] = fcn(q_c)
    qy = max(min(q_c(2), 1), -1);
    beta_c = asin(qy);
    alpha_c = atan2(q_c(1), -q_c(3));
end

== matlab function slide_mode_control/inner-loop controller/Subsystem/commanded filter1 ==
  data: phi_d input; dot_phi_d output; phi_d_f input; dot_phi_d_scaled input; zeta_2 parameter; ddot_phi_d_scaled output; omega_n_2 parameter
function [dot_phi_d, ddot_phi_d_scaled] = fcn(phi_d, phi_d_f, dot_phi_d_scaled, zeta_2, omega_n_2)
    dot_phi_d = omega_n_2 * dot_phi_d_scaled;
    ddot_phi_d_scaled = -2 * zeta_2 * omega_n_2 * dot_phi_d_scaled - omega_n_2 * (phi_d_f - phi_d);
end

== matlab function slide_mode_control/Swing angle controller/commanded filter1 ==
  data: alp_d input; dot_alp_d output; alp_d_f input; dot_alp_d_scaled input; zeta_1 parameter; ddot_alp_d_scaled output; omega_n_1 parameter
function [dot_alp_d, ddot_alp_d_scaled] = fcn(alp_d, alp_d_f, dot_alp_d_scaled, zeta_1, omega_n_1)
    dot_alp_d = omega_n_1 * dot_alp_d_scaled;
    ddot_alp_d_scaled = -2 * zeta_1 * omega_n_1 * dot_alp_d_scaled - omega_n_1 * (alp_d_f - alp_d);
end

== matlab function slide_mode_control/target attitude calculation ==
  data: u_tot_x input; phi_d output; u_tot_y input; psi_d input; theta_d output
function [phi_d, theta_d] = fcn(u_tot_x, u_tot_y, psi_d)

term_1=sin(psi_d)*u_tot_x-cos(psi_d)*u_tot_y;
term_2=min(max(term_1,-1),1);
phi_d=asin(term_2);

cos_phi=max(cos(phi_d), 1e-3);

term_3=(cos(psi_d) * u_tot_x + sin(psi_d) * u_tot_y) / cos_phi;
term_4=min(max(term_3,-1),1);
theta_d=asin(term_4);
    
   
end

== matlab function slide_mode_control/Swing angle controller/commanded filter2 ==
  data: beta_d input; dot_beta_d output; beta_d_f input; dot_beta_d_scaled input; zeta_2 parameter; ddot_beta_d_scaled output; omega_n_2 parameter
function [dot_beta_d, ddot_beta_d_scaled] = fcn(beta_d, beta_d_f, dot_beta_d_scaled, zeta_2, omega_n_2)
    dot_beta_d = omega_n_2 * dot_beta_d_scaled;
    ddot_beta_d_scaled = -2 * zeta_2 * omega_n_2 * dot_beta_d_scaled - omega_n_2 * (beta_d_f - beta_d);
end

== matlab function slide_mode_control/inner-loop controller/MATLAB Function ==
  data: u_2 output; u_3 output; u_4 output; phi input; theta input; psi input; d_phi input; d_theta input; d_psi input; phi_d input; theta_d input; psi_d input; d_phi_d input; d_theta_d input; d_psi_d input; dd_phi_d input; dd_theta_d input; dd_psi_d input; Omega input; Ixx parameter; J_rp parameter; Iyy parameter; Izz parameter; c1_inner parameter; c2_inner parameter; k_inner parameter; mu_1_inner parameter; mu_2_inner parameter; epn_inner parameter; delta_val parameter
function [u_2, u_3, u_4] = fcn(phi, theta, psi, d_phi, d_theta, d_psi, phi_d, theta_d, psi_d, ...
    d_phi_d, d_theta_d, d_psi_d, dd_phi_d, ...
    dd_theta_d, dd_psi_d, Omega, Ixx, J_rp, Iyy, Izz, c1_inner, c2_inner,k_inner,mu_1_inner,mu_2_inner,epn_inner,delta_val)

    e_phi   = phi_d - phi;
    e_theta = theta_d - theta;
    e_psi   = psi_d - psi;

    dot_e_phi   = d_phi_d - d_phi;
    dot_e_theta = d_theta_d - d_theta;
    dot_e_psi   = d_psi_d - d_psi;

    g_phi   = 1 / Ixx;
    g_theta = 1 / Iyy;
    g_psi   = 1 / Izz;

    f_phi   = d_theta * d_psi * (Iyy - Izz) + J_rp * d_theta * Omega;
    f_theta = d_phi * d_psi * (Izz - Ixx) + J_rp * d_phi * Omega;
    f_psi   = d_phi * d_theta * (Ixx - Iyy);

    % Surface parameters
    c1 = c1_inner; 
    c2 = c2_inner; 
    mu_1 = mu_1_inner; 
    mu_2 = mu_2_inner; 
    epn = epn_inner;


    s_phi   = e_phi   + c1 * sign(e_phi)   * abs(e_phi)^mu_1   + c2 * sign(dot_e_phi)   * abs(dot_e_phi)^mu_2;
    s_theta = e_theta + c1 * sign(e_theta) * abs(e_theta)^mu_1 + c2 * sign(dot_e_theta) * abs(dot_e_theta)^mu_2;
    s_psi   = e_psi   + c1 * sign(e_psi)   * abs(e_psi)^mu_1   + c2 * sign(dot_e_psi)   * abs(dot_e_psi)^mu_2;

    delta=delta_val;

    num2 = (sign(dot_e_phi) * abs(dot_e_phi)^(2-mu_2) / (c2 * mu_2)) * (1 + c1 * mu_1 * abs(e_phi)^(mu_1-1)) + dd_phi_d - f_phi + k_inner * s_phi + epn * sat(s_phi, delta);
    num3 = (sign(dot_e_theta) * abs(dot_e_theta)^(2-mu_2) / (c2 * mu_2)) * (1 + c1 * mu_1 * abs(e_theta)^(mu_1-1)) + dd_theta_d - f_theta + k_inner * s_theta + epn * sat(s_theta, delta);
    num4 = (sign(dot_e_psi) * abs(dot_e_psi)^(2-mu_2) / (c2 * mu_2)) * (1 + c1 * mu_1 * abs(e_psi)^(mu_1-1)) + dd_psi_d - f_psi + k_inner * s_psi + epn * sat(s_psi, delta);

    u_2 = num2 / g_phi;
    u_3 = num3 / g_theta;
    u_4 = num4 / g_psi;
end

== matlab function slide_mode_control/model/dynamics ==
  data: u_1 input; u_2 input; u_3 input; u_4 input; alpha input; beta input; d_alpha input; d_beta input; l input; d_l input; phi input; theta input; psi input; d_phi input; d_theta input; d_psi input; dd_alpha output; dd_beta output; dd_l output; dd_phi output; dd_theta output; dd_psi output; dd_x output; dd_y output; dd_z output; M parameter; k_plant parameter; c_plant parameter; L_rest parameter; m_plant parameter; Ixx parameter; Iyy parameter; Izz parameter; cT parameter; cM parameter; d parameter; J_rp parameter; Omega output; omega_square output
function [dd_alpha,dd_beta,dd_l,dd_phi,dd_theta,dd_psi,dd_x,dd_y,dd_z,Omega, omega_square]=dynamics(u_1,u_2,u_3,u_4,alpha, ...
    beta,d_alpha,d_beta,l,d_l,phi,theta,psi,d_phi,d_theta,d_psi,M, k_plant, c_plant, L_rest, ...
    m_plant, Ixx, Iyy, Izz, cT, cM, d, J_rp)

l_safe = max(l, 0.05);
cos_beta_safe = max(cos(beta), 0.05);
g=9.81;
T=k_plant*(l-L_rest)+c_plant*d_l;
a=sqrt(2)/2;
A=[cT cT cT cT;-a*d*cT a*d*cT a*d*cT -a*d*cT;-a*d*cT -a*d*cT a*d*cT a*d*cT;-cM cM -cM cM];
omega_square= inv(A)*[u_1;u_2;u_3;u_4];
w1 = sqrt(max(0, omega_square(1)));
w2 = sqrt(max(0, omega_square(2)));
w3 = sqrt(max(0, omega_square(3)));
w4 = sqrt(max(0, omega_square(4)));

Omega = w1 - w2 + w3 - w4;

Fx = u_1 * (cos(psi)*sin(theta)*cos(phi) + sin(psi)*sin(phi));
Fy = u_1 * (sin(psi)*sin(theta)*cos(phi) - cos(psi)*sin(phi));
Fz = u_1 * (cos(theta)*cos(phi));

dd_alpha=-(Fx/(M*l_safe))*(cos(alpha)/cos_beta_safe)-(Fz/(M*l_safe))*(sin(alpha)/cos_beta_safe)-2*d_l*d_alpha/l_safe+2*d_alpha*d_beta*(sin(beta)/cos_beta_safe);
dd_beta=(Fx/(M*l_safe))*sin(alpha)*sin(beta)-(Fy/(M*l_safe))*cos(beta)-(Fz/(M*l_safe))*cos(alpha)*sin(beta)-2*d_l*d_beta/l_safe-d_alpha^2*sin(beta)*cos(beta);
dd_l=-(Fx/M)*sin(alpha)*cos(beta)-(Fy/M)*sin(beta)+(Fz/M)*cos(alpha)*cos(beta)-T*((1/m_plant)+(1/M))+l*d_beta^2+l*d_alpha^2*(cos(beta))^2;

dd_phi=(1/Ixx)*(u_2+d_theta*d_psi*(Iyy-Izz)+J_rp*d_theta*Omega);
dd_theta=(1/Iyy)*(u_3+d_phi*d_psi*(Izz-Ixx)+J_rp*d_phi*Omega);
dd_psi=(1/Izz)*(u_4+d_phi*d_theta*(Ixx-Iyy));

dd_x=(Fx/M)-(T/M)*sin(alpha)*cos(beta);
dd_y=(Fy/M)-(T/M)*sin(beta);
dd_z=(Fz/M)-(T/M)*cos(alpha)*cos(beta)-g;



end
